simulink model "Two_Stage_NIBB_Shared_Boost_data"  (R2022a)
settings: Solver=ode23tb  StartTime=0.0  StopTime=0.5  FixedStep=2e-7
libraries: spsSeriesRLCBranchLib x4, spsMosfetLib x3, simulink x3, spsDiodeLib x3, spsCurrentMeasurementLib x2, spsMeanLib x2, eePowerMeasurement x2, spsVoltageMeasurementLib x2, spsDCVoltageSourceLib x1, spsMultimeterLib x1, spspowerguiLib x1
settings Model: SimulationMode=accelerator  Creator=Bobby  LastModifiedBy=Bobby
settings DataIOCC: ReturnWorkspaceOutputs=off

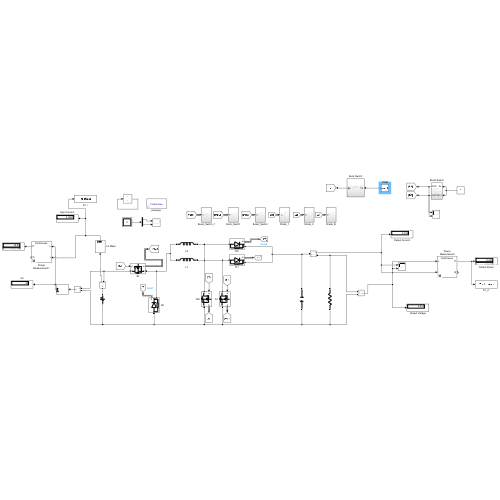
[thumbnail: Simulink's stored preview of the top-level diagram]
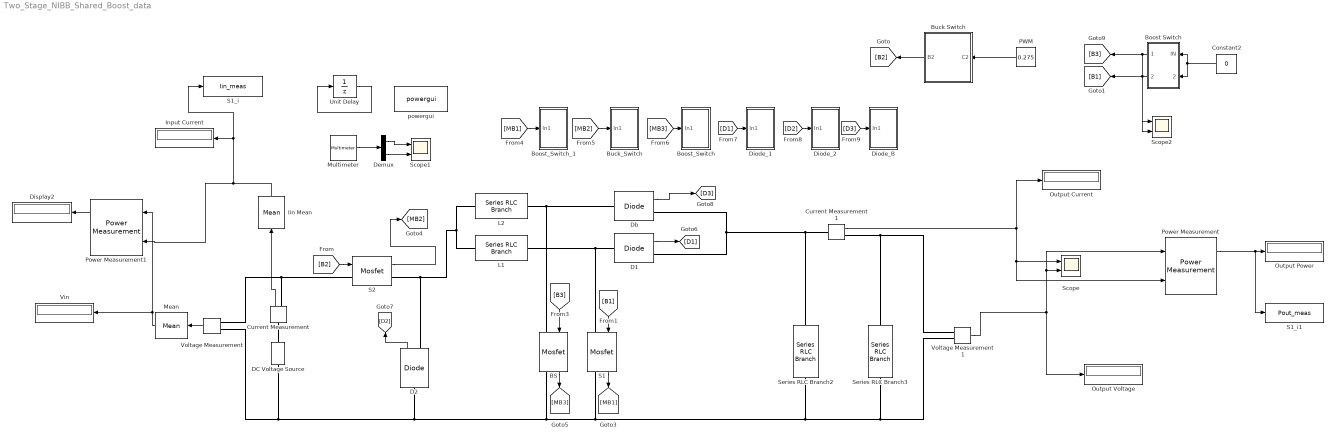
== system Two_Stage_NIBB_Shared_Boost_data ==
  BS : spsMosfetLib/Mosfet  Ron=0.1  Lon=0  Rd=0.01  Vfd=0  IC=0  Rs=1e5  Cs=inf  Measurements=on
  Boost Switch : Subsystem
  Boost_Switch : Subsystem
  Boost_Switch_1 : Subsystem
  Buck Switch : Subsystem
  Buck_Switch : Subsystem
  Constant2 : Constant  Value=0
  Current Measurement : spsCurrentMeasurementLib/Current Measurement  PhasorSimulation=off  OutputType=Complex  PSBequivalent=0
  Current Measurement1 : spsCurrentMeasurementLib/Current Measurement  PhasorSimulation=off  OutputType=Complex  PSBequivalent=0
  D1 : spsDiodeLib/Diode  Ron=0.001  Lon=0  Vf=0.8  IC=0  UseSnubber=0  Rs=500  Cs=250e-9  Measurements=on
  D2 : spsDiodeLib/Diode  Ron=0.001  Lon=0  Vf=0.8  IC=0  UseSnubber=0  Rs=500  Cs=250e-9  Measurements=on
  DC Voltage Source : spsDCVoltageSourceLib/DC Voltage Source  Amplitude=48  Measurements=None
  Db : spsDiodeLib/Diode  Ron=0.001  Lon=0  Vf=0.8  IC=0  UseSnubber=0  Rs=500  Cs=250e-9  Measurements=on
  Demux : Demux  Outputs=2
  Diode_1 : Subsystem
  Diode_2 : Subsystem
  Diode_B : Subsystem
  Display2 : Display
  Iin Mean : spsMeanLib/Mean  Freq=60  Vinit=0  Ts=0
  Input Current : Display
  L1 : spsSeriesRLCBranchLib/Series RLC Branch  LConnTagsString=__new0  RConnTagsString=__new0  BranchType=L  Resistance=1  Inductance=200e-6  SetiL0=off  InitialCurrent=0  Capacitance=1e-6  Setx0=off  InitialVoltage=0  Measurements=Branch current
  L2 : spsSeriesRLCBranchLib/Series RLC Branch  LConnTagsString=__new0  RConnTagsString=__new0  BranchType=L  Resistance=1  Inductance=200e-6  SetiL0=off  InitialCurrent=0  Capacitance=1e-6  Setx0=off  InitialVoltage=0  Measurements=Branch current
  Mean : spsMeanLib/Mean  Freq=60  Vinit=0  Ts=0
  Multimeter : spsMultimeterLib/Multimeter  L=2  sel=[1 2]  yselected={}  Gain=[1 1]  OutputType=Complex  PlotAtSimulationStop=off  PhasorSimulation=off
  Output Current : Display
  Output Power : Display
  Output Voltage : Display
  PWM : Constant  Value=0.275
  Power Measurement : eePowerMeasurement/Power Measurement  LabelModeActiveChoice=Continuous  F=60  K=[0 1 2 3]  Ts=0
      settings: SourceProductBaseCode=PS
  Power Measurement1 : eePowerMeasurement/Power Measurement  LabelModeActiveChoice=Continuous  F=60  K=[0 1 2 3]  Ts=0
      settings: SourceProductBaseCode=PS
  S1 : spsMosfetLib/Mosfet  Ron=0.1  Lon=0  Rd=0.01  Vfd=0  IC=0  Rs=1e5  Cs=inf  Measurements=on
  S1_i : ToWorkspace  VariableName=Iin_meas  SampleTime=-1
      settings: Save2DSignal=2-D array (concatenate along first dimension)
  S1_i1 : ToWorkspace  VariableName=Pout_meas  SampleTime=-1
      settings: Save2DSignal=2-D array (concatenate along first dimension)
  S2 : spsMosfetLib/Mosfet  Ron=0.1  Lon=0  Rd=0.01  Vfd=0  IC=0  Rs=1e5  Cs=inf  Measurements=on
  Scope : Scope  NumInputPorts=2
  Scope1 : Scope  NumInputPorts=2
  Scope2 : Scope  NumInputPorts=2
  Series RLC Branch2 : spsSeriesRLCBranchLib/Series RLC Branch  LConnTagsString=__new0  RConnTagsString=__new0  BranchType=C  Resistance=1  Inductance=1e-3  SetiL0=off  InitialCurrent=0  Capacitance=1666e-6  Setx0=off  InitialVoltage=0  Measurements=None
  Series RLC Branch3 : spsSeriesRLCBranchLib/Series RLC Branch  LConnTagsString=__new0  RConnTagsString=__new0  BranchType=R  Resistance=0.576  Inductance=1e-3  SetiL0=off  InitialCurrent=0  Capacitance=1e-6  Setx0=off  InitialVoltage=0  Measurements=None
  Unit Delay : UnitDelay  SampleTime=-1  HasFrameUpgradeWarning=on
  Vin : Display
  Voltage Measurement : spsVoltageMeasurementLib/Voltage Measurement  PhasorSimulation=off  OutputType=Complex  PSBequivalent=0
  Voltage Measurement1 : spsVoltageMeasurementLib/Voltage Measurement  PhasorSimulation=off  OutputType=Complex  PSBequivalent=0
  powergui : spspowerguiLib/powergui  Priority=1  SimulationMode=Continuous  SampleTime=50e-6  frequency=60  Iterations=50  frequencyindice=0  Pbase=100e6  ErrMax=1e-4  UnitsV=kV  UnitsW=MW  buscounter=0  FunctionMessages=off  echomessages=off  EnableUseOfTLC=off  CurrentSourceSwitches=off  DisableSnubberDevices=off  DisableRonSwitches=off  DisableVfSwitches=off  DisplayEquations=off  AutomaticDiscreteSolvers=off  SolverType=Tustin/Backward Euler (TBE)  Interpol=off  ExternalGateDelay=off  methode=off  Ts=100  x0status=blocks  SPID=on  SwTol=0  HookPort=off  NonlinearTolerance=1e-4  nMaxIteration=100  ContinueOnMaxIteration=off  RestoreLinks=warning  ResistiveCurrentMeasurement=off  Frange=[0:2:500]  Ylog=off  Xlog=on  ShowGrid=off  save=off  variable=ZData  structure=0  ZoomFFT=off  StartTime=0.0  cycles=1  DisplayStyle=1  fundamental=60  FreqAxis=off  MaxFrequency=1000  frequencyindicesteady=1  RmsSteady=1  display=off
  wires:
  Current Measurement1/1 -> Output Current/1, Power Measurement/2, Scope/1
  Voltage Measurement1/1 -> Power Measurement/1, Scope/2, Output Voltage/1
  Power Measurement/1 -> S1_i1/1, Output Power/1
  Voltage Measurement/1 -> Mean/1
  Current Measurement/1 -> Iin Mean/1
  Mean/1 -> Vin/1, Power Measurement1/1
  Iin Mean/1 -> S1_i/1, Input Current/1, Power Measurement1/2
  Power Measurement1/1 -> Display2/1
  Unit Delay/1 -> Unit Delay/1
  Multimeter/1 -> Demux/1
  Demux/2 -> Scope1/2
  Demux/1 -> Scope1/1
  Constant2/1 -> Boost Switch/1("IN "), Boost Switch/2(IN 1)
  PWM/1 -> Buck Switch/1(C2)
  [B2] -> S2/1
  [B1] -> S1/1
  Buck Switch/1(B2) -> [B2]
  Boost Switch/2(OUT1) -> Scope2/1, [B1]
  S1/1 -> [MB1]
  S2/1 -> [MB2]
  BS/1 -> [MB3]
  D1/1 -> [D1]
  D2/1 -> [D2]
  Db/1 -> [D3]
  Boost Switch/1(OUT) -> Scope2/2, [B3]
  [B3] -> BS/1
  [D3] -> Diode_B/1(In1)
  [MB2] -> Buck_Switch/1(In1)
  [D2] -> Diode_2/1(In1)
  [MB1] -> Boost_Switch_1/1(In1)
  [D1] -> Diode_1/1(In1)
  [MB3] -> Boost_Switch/1(In1)
  connections:
  Current Measurement/LConn1 -- DC Voltage Source/RConn1
  Current Measurement/RConn1 -- Voltage Measurement/LConn1 -- S2/LConn1
  D2/LConn1 -- Voltage Measurement1/LConn2 -- Series RLC Branch3/RConn1 -- Series RLC Branch2/RConn1 -- S1/RConn1 -- BS/RConn1 -- Voltage Measurement/LConn2 -- DC Voltage Source/LConn1
  Series RLC Branch3/LConn1 -- Voltage Measurement1/LConn1 -- Current Measurement1/RConn1
  L2/RConn1 -- BS/LConn1 -- Db/LConn1
  D1/LConn1 -- L1/RConn1 -- S1/LConn1
  Db/RConn1 -- Current Measurement1/LConn1 -- Series RLC Branch2/LConn1 -- D1/RConn1
  L1/LConn1 -- S2/RConn1 -- D2/RConn1 -- L2/LConn1

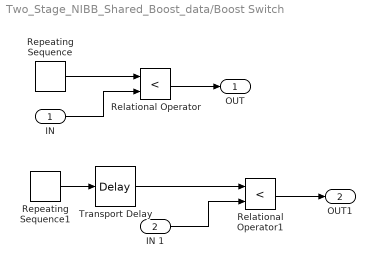
== system Two_Stage_NIBB_Shared_Boost_data/Boost Switch ==
  "IN " : Inport
  IN 1 : Inport  Port=2
  Relational Operator : RelationalOperator  Operator=<  OutDataTypeStr=boolean  RndMeth=Simplest  InputSameDT=off
  Relational Operator1 : RelationalOperator  Operator=<  OutDataTypeStr=boolean  RndMeth=Simplest  InputSameDT=off
  Repeating Sequence : simulink/Sources/Repeating Sequence  rep_seq_t=[0, 1e-5, 2e-5]  rep_seq_y=[0 1 0]
  Repeating Sequence1 : simulink/Sources/Repeating Sequence  rep_seq_t=[0, 1e-5, 2e-5]  rep_seq_y=[0 1 0]
  Transport Delay : TransportDelay  DelayTime=10e-6
  OUT : Outport
  OUT1 : Outport  Port=2
  wires:
  Repeating Sequence/1 -> Relational Operator/1
  "IN "/1 -> Relational Operator/2
  Relational Operator/1 -> OUT/1
  Relational Operator1/1 -> OUT1/1
  Repeating Sequence1/1 -> Transport Delay/1
  IN 1/1 -> Relational Operator1/2
  Transport Delay/1 -> Relational Operator1/1

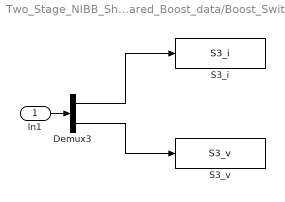
== system Two_Stage_NIBB_Shared_Boost_data/Boost_Switch ==
  In1 : Inport
  Demux3 : Demux  Outputs=2
  S3_i : ToWorkspace  VariableName=S3_i  SampleTime=-1
      settings: Save2DSignal=2-D array (concatenate along first dimension)
  S3_v : ToWorkspace  VariableName=S3_v  SampleTime=-1
      settings: Save2DSignal=2-D array (concatenate along first dimension)
  wires:
  Demux3/2 -> S3_v/1
  Demux3/1 -> S3_i/1
  In1/1 -> Demux3/1

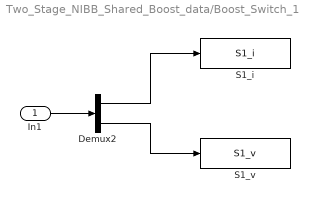
== system Two_Stage_NIBB_Shared_Boost_data/Boost_Switch_1 ==
  In1 : Inport
  Demux2 : Demux  Outputs=2
  S1_i : ToWorkspace  VariableName=S1_i  SampleTime=-1
      settings: Save2DSignal=2-D array (concatenate along first dimension)
  S1_v : ToWorkspace  VariableName=S1_v  SampleTime=-1
      settings: Save2DSignal=2-D array (concatenate along first dimension)
  wires:
  In1/1 -> Demux2/1
  Demux2/2 -> S1_v/1
  Demux2/1 -> S1_i/1

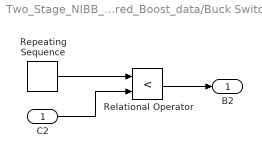
== system Two_Stage_NIBB_Shared_Boost_data/Buck Switch ==
  C2 : Inport
  Relational Operator : RelationalOperator  Operator=<  OutDataTypeStr=boolean  RndMeth=Simplest  InputSameDT=off
  Repeating Sequence : simulink/Sources/Repeating Sequence  rep_seq_t=[0, 1e-5, 2e-5]  rep_seq_y=[0 1 0]
  B2 : Outport
  wires:
  Repeating Sequence/1 -> Relational Operator/1
  C2/1 -> Relational Operator/2
  Relational Operator/1 -> B2/1

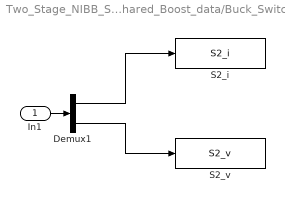
== system Two_Stage_NIBB_Shared_Boost_data/Buck_Switch ==
  In1 : Inport
  Demux1 : Demux  Outputs=2
  S2_i : ToWorkspace  VariableName=S2_i  SampleTime=-1
      settings: Save2DSignal=2-D array (concatenate along first dimension)
  S2_v : ToWorkspace  VariableName=S2_v  SampleTime=-1
      settings: Save2DSignal=2-D array (concatenate along first dimension)
  wires:
  Demux1/2 -> S2_v/1
  Demux1/1 -> S2_i/1
  In1/1 -> Demux1/1

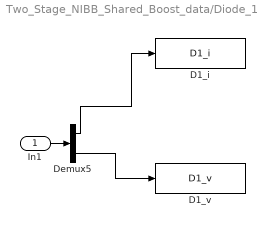
== system Two_Stage_NIBB_Shared_Boost_data/Diode_1 ==
  In1 : Inport
  D1_i : ToWorkspace  VariableName=D1_i  SampleTime=-1
      settings: Save2DSignal=2-D array (concatenate along first dimension)
  D1_v : ToWorkspace  VariableName=D1_v  SampleTime=-1
      settings: Save2DSignal=2-D array (concatenate along first dimension)
  Demux5 : Demux  Outputs=2
  wires:
  Demux5/2 -> D1_v/1
  Demux5/1 -> D1_i/1
  In1/1 -> Demux5/1

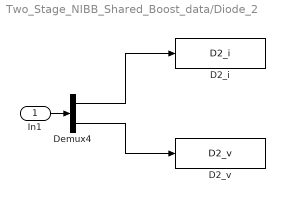
== system Two_Stage_NIBB_Shared_Boost_data/Diode_2 ==
  In1 : Inport
  D2_i : ToWorkspace  VariableName=D2_i  SampleTime=-1
      settings: Save2DSignal=2-D array (concatenate along first dimension)
  D2_v : ToWorkspace  VariableName=D2_v  SampleTime=-1
      settings: Save2DSignal=2-D array (concatenate along first dimension)
  Demux4 : Demux  Outputs=2
  wires:
  Demux4/2 -> D2_v/1
  Demux4/1 -> D2_i/1
  In1/1 -> Demux4/1

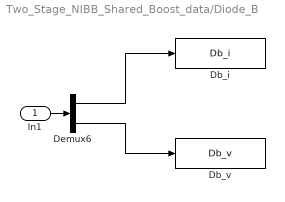
== system Two_Stage_NIBB_Shared_Boost_data/Diode_B ==
  In1 : Inport
  Db_i : ToWorkspace  VariableName=Db_i  SampleTime=-1
      settings: Save2DSignal=2-D array (concatenate along first dimension)
  Db_v : ToWorkspace  VariableName=Db_v  SampleTime=-1
      settings: Save2DSignal=2-D array (concatenate along first dimension)
  Demux6 : Demux  Outputs=2
  wires:
  In1/1 -> Demux6/1
  Demux6/2 -> Db_v/1
  Demux6/1 -> Db_i/1
